simulink model "AM"  (R2023b)
settings: Solver=VariableStepAuto  StartTime=0.0  StopTime=1  RelTol=1e-3
libraries: commanapbnd3 x1
settings Model: Creator=lxl  LastModifiedBy=lxl

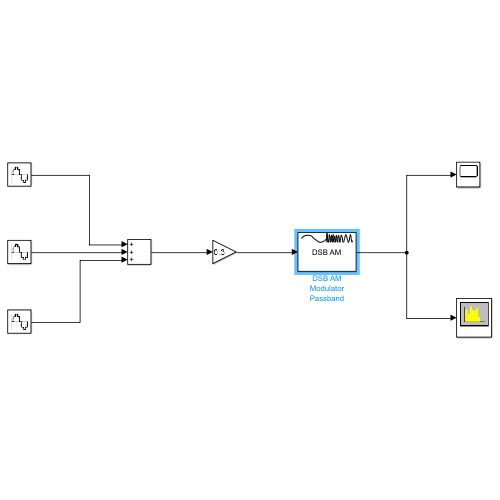
[thumbnail: Simulink's stored preview of the top-level diagram]
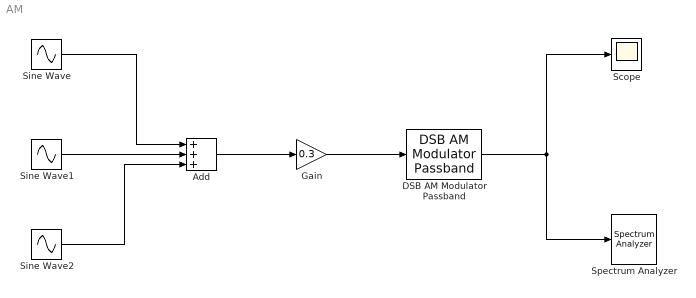
== system AM ==
  Add : Sum  Inputs=+++
  DSB AM Modulator Passband : commanapbnd3/DSB AM Modulator Passband  Fc=500  Ph=0  Offset=5
  Gain : Gain  Gain=0.3
  Scope : Scope
  Sine Wave : Sin  Amplitude=0.3  Frequency=2*pi*10  SampleTime=1/3000
  Sine Wave1 : Sin  Amplitude=0.2  Frequency=2*pi*20  Phase=pi/6  SampleTime=1/3000
  Sine Wave2 : Sin  Amplitude=0.5  Frequency=2*pi*30  Phase=pi/3  SampleTime=1/3000
  Spectrum Analyzer : SpectrumAnalyzer  WindowPosition=[368.000000,182.000000,800.000000,500.000000,]  ScopeFrameLocation=window  Span=3000  StartFrequency=-1500  StopFrequency=1500  YLimits=[-167.85497226,-49.71476188]
  wires:
  Sine Wave/1 -> Add/1
  Sine Wave1/1 -> Add/2
  Sine Wave2/1 -> Add/3
  Add/1 -> Gain/1
  Gain/1 -> DSB AM Modulator Passband/1
  DSB AM Modulator Passband/1 -> Spectrum Analyzer/1, Scope/1
